simulink model "afe_dqctrl_inv_psm"  (R2026a)
settings: Solver=ode23t  StopTime=simlength  FixedStep=tc  MaxStep=glb_time.tc  RelTol=1e-4
values from neighbouring files (symbols this model uses):
  afe_ctrl = ctrl_afe_setup(glb_time.ts_afe, grid_emu.omega_grid_nom)    [init_model.m]
  afe_pwm_phase_shift_mod1 = 0    [init_model.m]
  CTRPIFF_CLIP_RELEASE = 0.001    [init_model.m]
  filters = setup_global_filters(glb_time.ts_afe, glb_time.ts_inv, glb_time.ts_dab, glb_time.tc)    [init_model.m]
  glb_time = timing_setup(fpwm_afe, trgo_afe, fpwm_inv, trgo_inv, fpwm_single_phase_inv, trgo_single_phase_inv, fpwm_dab, trgo_dab,      fpwm_psfbc, trgo_psfbc, fpwm_isop_rail, trgo_isop_rail, fpwm_cllc, trgo_cllc, t_measure, tc_factor, tc_decimation, delay_pwm, dead_time_afe,      dead_time_inv, dead_time_single_phase_inv, dead_time_dab, dead_time_psfbc, dead_time_isop_rail, dead_time_cllc)    [init_model.m]
  grid_emu = grid_three_phase_emulator('Dyn11', delta_star, grid_nominal_power, application_voltage, us1, us2, fgrid,                  eq_grid_inductance, eq_grid_resistance, eta, ucc, i1m, p_iron, n1, n2, core_area, core_length, mur,                  up_xi_pu_ref, up_eta_pu_ref, un_xi_pu_ref, un_eta_pu_ref)    [init_model.m]
  heatsink = liquid_cooled_plate_2kw_setup(weight, no_weight, cp_al, heat_capacity_hs, thermal_conductivity_al,      Rth_switch_HA, Rth_mosfet_HA, Rth_diode_HA, Tambient, DThs_init)    [init_model.m]
  inv_pwm_phase_shift_mod1 = 0    [init_model.m]
  ki_align = 18    [init_model.m]
  kp_align = 0.25    [init_model.m]
  lim_down_align = -0.05    [init_model.m]
  lim_up_align = 0.05    [init_model.m]
  omega_m_sim = psm.omega_m_bez    [init_model.m]
  psm = psm_calculus()    [init_model.m]
  psm_ctrl = ctrl_pmsm_setup(glb_time.ts_inv, psm.omega_bez, u_psm_scale, psm.Jm_norm)    [init_model.m]
  simlength = 1.75    [init_model.m]
  Tambient = 40    [init_model.m]
  time_gain_afe_module_1 = 1.0002    [init_model.m]
  time_gain_inv_module_2 = 1.001    [init_model.m]
  time_start_motor_control = 0.25    [init_model.m]
  torque_overload_factor = 1.15    [init_model.m]
  u_cm_comp_mod1 = 0    [init_model.m]
  u_psm_scale_ekf = sqrt(3)/2 * 2/3 * hwdata.inv.udc_nom/psm.ubez    [init_model.m]
undefined symbols (not defined in the file or in its folder): hwdata, igbt, magnitude, omega_m_bez, rpm_base, torque_base
libraries: fl_lib x99, nesl_utility x96, igbt_simple_lib x12, single_phase_transformer_lib x3, threephase_inductor_lib x2, dclink_for_two_levels x2, three_phase_pwm_modulator x2, cstblocks_lti x2, discrete_time_low_pass_filter x1, lithium_ion_battery x1, three_phase_voltage_with_frt_emulator x1, simple_flexible_shaft x1
(part 1 of 9)
settings Model: Creator=dbagn  LastModifiedBy=d.bagnara
settings SolverCC: NumberNewtonIterations=3.0  ZeroCrossControl=DisableAll  SolverResetMethod=Robust
settings SFSimCC: CustomCodeUndefinedFunction=ThrowError  DefaultCustomCodeDeterministicFunctions=All
settings SFSimCC: SimCustomHeaderCode=|
  | #include "rpi.h"
  | #include "rpi_simulink.h"
  | #include "bemf_obsv_load_est.h"
  | #include "bemf_obsv_load_est_simulink.h"
  | #include "dqpll_grid.h"
  | #include "dsmavgflt.h"
  | #include "bemf_obsv.h"
  | #include "bemf_obsv_simulink.h"
  | #include "mavgflt.h"
  | #include "mavgflt_simulink.h"
  | #include "mavgflts.h"
  | #include "mavgflts_simulink.h"
  | #include "sv_pwm_cm.h"
  | #include "dsmavgflt_simulink.h"
  | #include "linear_double_integrator_observer_simulink.h"
  | #include "sv_pwm_cm_simulink.h"
  | #include "dqvector_pi.h"
  | #include "dqpll_grid_simulink.h"
  | #include "first_harmonic_tracker.h"
  | #include "dqvector_pi_simulink.h"
  | #include "first_harmonic_tracker_simulink.h"
  | #include "dqpll_thyr.h"
  | #include "sv_pwm_simulink.h"
  | #include "sv_pwm.h"
  | #include "dqpll_thyr_simulink.h"
  | #include "linear_double_integrator_observer.h"
  | #include "math_f.h"
settings SFSimCC: SimUserSources=|
  | "rpi.c"
  | "rpi_simulink.c"
  | "mavgflt_simulink.c"
  | "mavgflt.c"
  | "mavgflts_simulink.c"
  | "mavgflts.c"
  | "dsmavgflt_simulink.c"
  | "dsmavgflt.c"
  | "bemf_obsv_simulink.c"
  | "bemf_obsv.c"
  | "bemf_obsv_load_est_simulink.c"
  | "bemf_obsv_load_est.c"
  | "dqvector_pi.c"
  | "dqvector_pi_simulink.c"
  | "sv_pwm_simulink.c"
  | "sv_pwm.c"
  | "first_harmonic_tracker_simulink.c"
  | "first_harmonic_tracker.c"
  | "dqpll_thyr_simulink.c"
  | "dqpll_thyr.c"
  | "dqpll_grid_simulink.c"
  | "dqpll_grid.c"
  | "linear_double_integrator_observer_simulink.c"
  | "linear_double_integrator_observer.c"
  | "sv_pwm_cm_simulink.c"
  | "sv_pwm_cm.c"
settings SFSimCC: SimUserIncludeDirs=|
  | include
  | src
settings SimscapeCC: SimscapeNominalValues="[{\"value\":\"1\",\"unit\":\"A\"},{\"value\":\"1\",\"unit\":\"bar\"},{\"value\":\"1\",\"unit\":\"cm^2\"},{\"value\":\"1\",\"unit\":\"cm^3/s\"},{\"value\":\"1\",\"unit\":\"kJ/kg\"},{\"value\":\"1\",\"unit\":\"kW\"},{\"value\":\"1\",\"unit\":\"l\"},{\"value\":\"1\",\"unit\":\"N\"},{\"value\":\"1\",\"unit\":\"N*m\"},{\"value\":\"1\",\"unit\":\"V\"}]"  SimscapeLogType=none  SimscapeLogDataHistory=5000.0

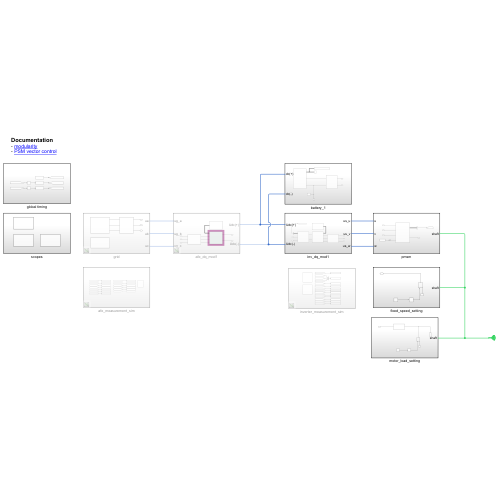
[thumbnail: Simulink's stored preview of the top-level diagram]
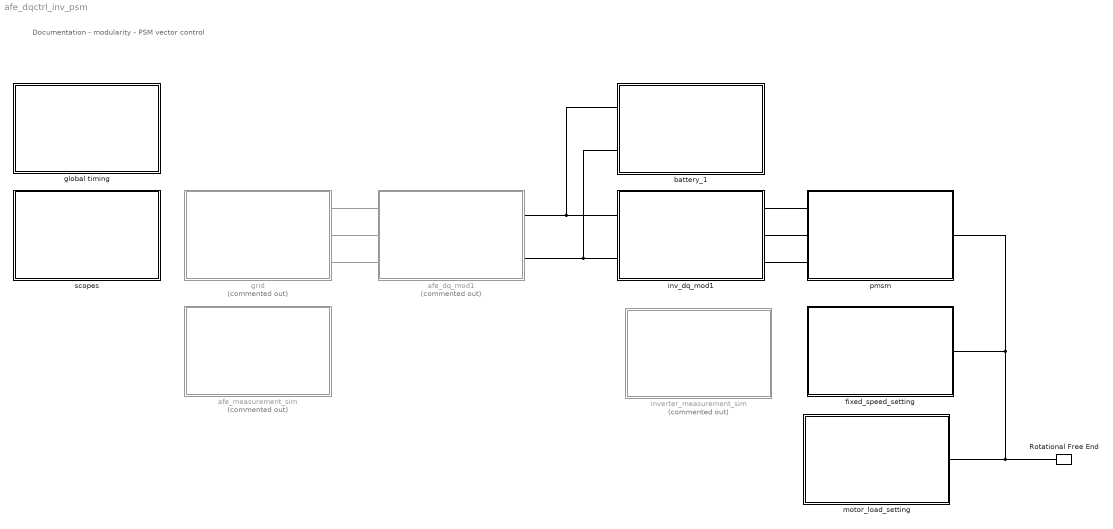
== system afe_dqctrl_inv_psm ==
  note: Documentation
      | - modularity
      | - PSM vector control
  Rotational Free End : fl_lib/Mechanical/Rotational Elements/Rotational Free End  w_specify=off  w_priority=None  w=0 rad/s  w_nominal_specify=off  w_nominal_value=1  w_nominal_unit=rad/s
  afe_dq_mod1 : Subsystem  Commented=on
  afe_measurement_sim : Subsystem  Commented=on
  battery_1 : Subsystem
  fixed_speed_setting : Subsystem
  global timing : Subsystem
  grid : Subsystem  Commented=on
  inv_dq_mod1 : Subsystem
  inverter_measurement_sim : Subsystem  Commented=on
  motor_load_setting : Subsystem
  pmsm : Subsystem
  scopes : Subsystem
  connections:
  pmsm/RConn1 -- motor_load_setting/LConn1 -- Rotational Free End/LConn1 -- fixed_speed_setting/LConn1
  afe_dq_mod1/LConn1 -- grid/RConn1
  afe_dq_mod1/LConn3 -- grid/RConn3
  afe_dq_mod1/LConn2 -- grid/RConn2
  inv_dq_mod1/RConn2 -- pmsm/LConn2
  inv_dq_mod1/RConn1 -- pmsm/LConn1
  inv_dq_mod1/RConn3 -- pmsm/LConn3
  inv_dq_mod1/LConn1 -- afe_dq_mod1/RConn1 -- battery_1/RConn1
  inv_dq_mod1/LConn2 -- afe_dq_mod1/RConn2 -- battery_1/RConn2

== system afe_dqctrl_inv_psm/afe_dq_mod1 ==
  AFE_control : Subsystem
  LCL_filter : Subsystem
  afe : Subsystem
  ug_a : PMIOPort  Side=Left
  ug_b : PMIOPort  Port=2  Side=Left
  ug_c : PMIOPort  Port=3  Side=Left
  Udc(+) : PMIOPort  Port=4  Side=Right
  Udc(-) : PMIOPort  Port=5  Side=Right
  wires:
  AFE_control/1(dabc_out) -> afe/1(dabc)
  connections:
  Udc(-)/RConn1 -- afe/RConn2
  Udc(+)/RConn1 -- afe/RConn1
  LCL_filter/LConn1 -- afe/LConn1
  LCL_filter/LConn2 -- afe/LConn2
  LCL_filter/LConn3 -- afe/LConn3
  ug_a/RConn1 -- LCL_filter/RConn1
  ug_b/RConn1 -- LCL_filter/RConn2
  ug_c/RConn1 -- LCL_filter/RConn3

== system afe_dqctrl_inv_psm/afe_measurement_sim ==
  From6 : From  Commented=on  GotoTag=ileg_dc_afe_mod1
  To Workspace : ToWorkspace  VariableName=t_tc_sim  SampleTime=glb_time.tc
      settings: MaxDataPoints=glb_time.Nc
  To Workspace10 : ToWorkspace  VariableName=P1n_sim  SampleTime=glb_time.ts_afe
      settings: MaxDataPoints=glb_time.Ns_afe
  To Workspace12 : ToWorkspace  Commented=on  VariableName=ileg_dc_afe_sim_mod1  SampleTime=glb_time.tc
      settings: MaxDataPoints=glb_time.Nc
  To Workspace2 : ToWorkspace  VariableName=ic_dclink_sim_mod1  SampleTime=glb_time.tc
      settings: MaxDataPoints=glb_time.Nc
  To Workspace22 : ToWorkspace  VariableName=ig_abc_sim  SampleTime=glb_time.tc
      settings: MaxDataPoints=glb_time.Nc
  To Workspace23 : ToWorkspace  VariableName=ug_abc_sim  SampleTime=glb_time.tc
      settings: MaxDataPoints=glb_time.Nc
  To Workspace3 : ToWorkspace  VariableName=udc_dclink_sim_mod1  SampleTime=glb_time.tc
      settings: MaxDataPoints=glb_time.Nc
  To Workspace4 : ToWorkspace  VariableName=ig_abc_sim_mod1  SampleTime=glb_time.tc
      settings: MaxDataPoints=glb_time.Nc
  To Workspace5 : ToWorkspace  VariableName=vg_abc_sim_mod1  SampleTime=glb_time.tc
      settings: MaxDataPoints=glb_time.Nc
  To Workspace6 : ToWorkspace  VariableName=is_abc_sim_mod1  SampleTime=glb_time.tc
      settings: MaxDataPoints=glb_time.Nc
  To Workspace7 : ToWorkspace  VariableName=Q1n_sim  SampleTime=glb_time.ts_afe
      settings: MaxDataPoints=glb_time.Ns_afe
  To Workspace8 : ToWorkspace  VariableName=Q1p_sim  SampleTime=glb_time.ts_afe
      settings: MaxDataPoints=glb_time.Ns_afe
  To Workspace9 : ToWorkspace  VariableName=P1p_sim  SampleTime=glb_time.ts_afe
      settings: MaxDataPoints=glb_time.Ns_afe
  igbt_power_losses : Subsystem
  wires:
  [time_master] -> To Workspace/1
  [Q1n_global] -> To Workspace7/1
  [Q1p_global] -> To Workspace8/1
  [P1p_global] -> To Workspace9/1
  [P1n_global] -> To Workspace10/1
  [ug_abc] -> To Workspace23/1
  [ig_abc] -> To Workspace22/1
  [ug_abc_pu_mod1] -> To Workspace5/1
  [ig_abc_pu_mod1] -> To Workspace4/1
  From6/1 -> To Workspace12/1
  [udc_mod1] -> To Workspace3/1
  [ic_dclink_mod1] -> To Workspace2/1
  [is_abc_pu_mod1] -> To Workspace6/1

== system afe_dqctrl_inv_psm/battery_1 ==
  Electrical Reference : fl_lib/Electrical/Electrical Elements/Electrical Reference
  Solver Configuration : nesl_utility/Solver Configuration  PhysicalDomain=network_engine_domain  SubClassName=solver  LeftPortType=input  RightPortType=generic  Tones=[]  Harmonics=[]  SimulateNoise=off  Profile=off  UseLocalSampling=off  EnableSwitchedLinearOptims=on  FrequencyDomain=off  UseCCode=off  RelTol=0.001  AbsTol=0.001  MinStep=1e-09  ToWorkspace=off  RevertToSquareIcSolve=off  NumHomotopyIterations=100  PhasorMode=off  PhasorModeNumHarmonics=1  ConsistencySolver=NEWTON_FTOL  CanonicalOrdering=UNORDERED  OptimizeIntermediates=UNOPTIMIZED  IndexReductionMethod=DerivativeReplacement  DoDC=on  ResidualTolerance=1e-09  ConsistencyTolSource=GLOBAL  ConsistencyAbsTol=0.001  ConsistencyRelTol=0.001  ConsistencyTolFactor=0.001  UseLocalSolver=on  LocalSolverChoice=NE_BACKWARD_EULER_ADVANCER  ResolveIndetEquations=on  FunctionEvalNumThread=1  LocalSolverSampleTime=glb_time.tc  DoFixedCost=on  MaxNonlinIter=nonlinear_iterations  MaxModeIter=2  ComputeImpulses=off  ImpulseIterations=2  LinearAlgebra=auto  LinearAlgebraNumThread=0  EquationFormulation=NE_TIME_EF  DelaysMemoryBudget=1024  AutomaticFiltering=on  FilteringTimeConstant=0.001  PartitionStorageMethod=AS_NEEDED  PartitionMemoryBudget=1024  PartitionMethod=ROBUST  MultibodyUseLocalSolver=off  MultibodyLocalSolverChoice=ODE1  MultibodyLocalSolverSampleTime=0.001
  To Workspace14 : ToWorkspace  VariableName=battery_1_data_sim  SampleTime=glb_time.tc
      settings: MaxDataPoints=glb_time.Nc  Decimation=glb_time.decimation_tc
  lithium ion battery : Scope
      settings: ActiveDisplayYMinimum=-808.27997881012811  ActiveDisplayYMaximum=1287.7546757937268  DataLoggingVariableName=ScopeData3
  lithium_ion_battery : lithium_ion_battery/lithium_ion_battery  Q=lithium_ion_battery_1.Q  number_of_cells=lithium_ion_battery_1.number_of_cells  E_1=lithium_ion_battery_1.E_1  E0=lithium_ion_battery_1.E0  E1=lithium_ion_battery_1.E1  E2=lithium_ion_battery_1.E2  E3=lithium_ion_battery_1.E3  Elog=lithium_ion_battery_1.Elog  R0=lithium_ion_battery_1.R0  R1=lithium_ion_battery_1.R1  C1=lithium_ion_battery_1.C1  M=lithium_ion_battery_1.M  alpha=lithium_ion_battery_1.alpha  soc_init=lithium_ion_battery_1.soc_init  ts_battery=glb_time.ts_dab  q1Kalman=lithium_ion_battery_1.q1Kalman  q2Kalman=lithium_ion_battery_1.q2Kalman  q3Kalman=lithium_ion_battery_1.q3Kalman  rKalman=lithium_ion_battery_1.rKalman  tc=glb_time.tc  enable_white_noise_m=0
  single_phase_ui_measure : Subsystem
  dc(+) : PMIOPort  Side=Right
  dc(-) : PMIOPort  Port=2  Side=Right
  wires:
  lithium_ion_battery/1 -> To Workspace14/1, lithium ion battery/1
  connections:
  Solver Configuration/RConn1 -- lithium_ion_battery/RConn2 -- single_phase_ui_measure/LConn2 -- Electrical Reference/LConn1
  single_phase_ui_measure/RConn1 -- dc(+)/RConn1
  single_phase_ui_measure/LConn1 -- lithium_ion_battery/RConn1
  dc(-)/RConn1 -- single_phase_ui_measure/RConn2

== system afe_dqctrl_inv_psm/fixed_speed_setting ==
  Ideal Angular Velocity Source : fl_lib/Mechanical/Mechanical Sources/Ideal Angular Velocity Source
  Mechanical Rotational Reference : fl_lib/Mechanical/Rotational Elements/Mechanical Rotational Reference
  PS Step1 : fl_lib/Physical Signals/Sources/PS Step  step_time=0.025 s  initial_value=0 rpm  final_value=rpm_sim rpm
  PS Transfer Function : fl_lib/Physical Signals/Linear Operators/PS Transfer Function  transfer_function_type=foundation.enum.transfer_function_type.lag  T=0.1 s  T1=2 s  T2=1 s  reset_method=foundation.enum.IntegratorResetSpec.None  initial_condition_spec=foundation.enum.IntegratorICSpec.Internal  y0=0 rpm
  shaft : PMIOPort  Side=Left
  connections:
  Mechanical Rotational Reference/LConn1 -- Ideal Angular Velocity Source/RConn2
  PS Step1/RConn1 -- PS Transfer Function/LConn1
  PS Transfer Function/RConn1 -- Ideal Angular Velocity Source/RConn1
  Ideal Angular Velocity Source/LConn1 -- shaft/RConn1

== system afe_dqctrl_inv_psm/global timing ==
  Unit Delay : UnitDelay  SampleTime=glb_time.tc
  Unit Delay1 : UnitDelay  SampleTime=glb_time.tc
  time_afe1 : Subsystem  mask{k=time_gain_afe_module_1}
      mask prompts: k "Time Gain"
      mask Display:
      | disp('time-gen');
      | port_label('input', 1, 'crt');
      | port_label('output', 1, 'tout');
  time_afe3 : Subsystem  mask{k=1}
      mask prompts: k "Time Gain"
      mask Display:
      | disp('time-gen');
      | port_label('output', 1, 'tout');
  time_inv1 : Subsystem  mask{k=time_gain_inv_module_2}
      mask prompts: k "Time Gain"
      mask Display:
      | disp('time-gen');
      | port_label('input', 1, 'crt');
      | port_label('output', 1, 'tout');
  tag scope: time_afe_module_1=global, time_inv_module_1=global, time_master=global
  wires:
  time_afe1/1(Out1) -> [time_afe_module_1]
  time_inv1/1(Out1) -> [time_inv_module_1]
  time_afe3/1(Out1) -> [time_master]
  [local_time_corr_afe1] -> Unit Delay/1
  Unit Delay/1 -> time_afe1/1(correction_time)
  [local_time_corr_inv1] -> Unit Delay1/1
  Unit Delay1/1 -> time_inv1/1(correction_time)

== system afe_dqctrl_inv_psm/grid ==
  grid_emulator : Subsystem
  power meter iec mfunc : Subsystem
  threephase_vi_measures : Subsystem
  ua : PMIOPort  Side=Right
  ub : PMIOPort  Port=2  Side=Right
  uc : PMIOPort  Port=3  Side=Right
  connections:
  threephase_vi_measures/LConn3 -- grid_emulator/RConn3
  threephase_vi_measures/LConn1 -- grid_emulator/RConn1
  threephase_vi_measures/RConn2 -- ub/RConn1
  threephase_vi_measures/LConn2 -- grid_emulator/RConn2
  threephase_vi_measures/RConn1 -- ua/RConn1
  threephase_vi_measures/RConn3 -- uc/RConn1

== system afe_dqctrl_inv_psm/inv_dq_mod1 ==
  Bus Selector : BusSelector  OutputSignals=vdc_pu
  INV_control : Subsystem
  L_filter : Subsystem
  dclink1 : dclink_for_two_levels/dclink  Cdc=hwdata.afe.CFi  Rudc_measure=1e6  Vdc_scale=hwdata.afe.udc_nom
  inverter : Subsystem
  Udc(+) : PMIOPort  Side=Left
  us_u : PMIOPort  Port=2  Side=Right
  us_v : PMIOPort  Port=3  Side=Right
  Udc(-) : PMIOPort  Port=4  Side=Left
  us_w : PMIOPort  Port=5  Side=Right
  tag scope: udc_pu_inv_mod1=global
  wires:
  INV_control/1(duvw_out) -> inverter/1(duvw)
  Bus Selector/1 -> [udc_pu_inv_mod1]  "<vdc_pu>"
  dclink1/1 -> Bus Selector/1
  connections:
  inverter/LConn1 -- L_filter/RConn1
  L_filter/LConn3 -- us_w/RConn1
  inverter/LConn3 -- L_filter/RConn3
  inverter/LConn2 -- L_filter/RConn2
  L_filter/LConn2 -- us_v/RConn1
  L_filter/LConn1 -- us_u/RConn1
  dclink1/LConn1 -- inverter/RConn1
  dclink1/LConn2 -- inverter/RConn2
  Udc(+)/RConn1 -- dclink1/RConn1
  Udc(-)/RConn1 -- dclink1/RConn2

== system afe_dqctrl_inv_psm/inverter_measurement_sim ==
  Bus Creator : BusCreator  Inputs=3
  To Workspace1 : ToWorkspace  VariableName=ud_psm_sim  SampleTime=glb_time.tc
      settings: MaxDataPoints=glb_time.Nc
  To Workspace10 : ToWorkspace  VariableName=rpm_motor_sim  SampleTime=glb_time.tc
      settings: MaxDataPoints=glb_time.Nc
  To Workspace11 : ToWorkspace  VariableName=iuvw_psm_sim  SampleTime=glb_time.tc
      settings: MaxDataPoints=glb_time.Nc
  To Workspace13 : ToWorkspace  VariableName=theta_elec_psm_sim  SampleTime=glb_time.tc
      settings: MaxDataPoints=glb_time.Nc
  To Workspace2 : ToWorkspace  VariableName=uq_psm_sim  SampleTime=glb_time.tc
      settings: MaxDataPoints=glb_time.Nc
  To Workspace3 : ToWorkspace  VariableName=iq_psm_sim  SampleTime=glb_time.tc
      settings: MaxDataPoints=glb_time.Nc
  To Workspace4 : ToWorkspace  VariableName=id_psm_sim  SampleTime=glb_time.tc
      settings: MaxDataPoints=glb_time.Nc
  To Workspace5 : ToWorkspace  VariableName=inverter_voltage_ee_phase_u_sim  SampleTime=glb_time.tc
      settings: MaxDataPoints=glb_time.Nc
  To Workspace6 : ToWorkspace  VariableName=inverter_voltage_ee_phase_v_sim  SampleTime=glb_time.tc
      settings: MaxDataPoints=glb_time.Nc
  To Workspace7 : ToWorkspace  VariableName=psi_r_alpha_psm_sim  SampleTime=glb_time.tc
      settings: MaxDataPoints=glb_time.Nc
  To Workspace8 : ToWorkspace  VariableName=inverter_voltage_ee_phase_w_sim  SampleTime=glb_time.tc
      settings: MaxDataPoints=glb_time.Nc
  To Workspace9 : ToWorkspace  VariableName=psi_r_beta_psm_sim  SampleTime=glb_time.tc
      settings: MaxDataPoints=glb_time.Nc
  igbt_power_losses : Subsystem
  module_1 : Subsystem
  wires:
  [psi_r_alpha_psm] -> To Workspace7/1  "phi_r_alpha_pmsm"
  [psi_r_beta_psm] -> To Workspace9/1  "phi_r_beta_pmsm"
  [rpm_motor] -> To Workspace10/1
  [iv_psm] -> Bus Creator/2  "iv"
  [iw_psm] -> Bus Creator/3  "iw"
  [iu_psm] -> Bus Creator/1  "iu"
  Bus Creator/1 -> To Workspace11/1
  [theta_elec_psm] -> To Workspace13/1  "theta_elec_pmsm"
  [ud_psm] -> To Workspace1/1  "ud_psm"
  [uq_psm] -> To Workspace2/1  "uq_psm"
  [iq_psm] -> To Workspace3/1  "iq_psm"
  [id_psm] -> To Workspace4/1  "id_psm"
  [inverter_voltage_ee_phase_u] -> To Workspace5/1
  [inverter_voltage_ee_phase_v] -> To Workspace6/1
  [inverter_voltage_ee_phase_w] -> To Workspace8/1

== system afe_dqctrl_inv_psm/motor_load_setting ==
  Ideal Torque Source : fl_lib/Mechanical/Mechanical Sources/Ideal Torque Source
  Inertia : fl_lib/Mechanical/Rotational Elements/Inertia  inertia=external_load_inertia kg*m^2  num_ports=foundation.enum.numPorts2.one  w_specify=off  w_priority=High  w=0 rad/s  w_nominal_specify=off  w_nominal_value=1  w_nominal_unit=rad/s  t_specify=off  t_priority=None  t=0 N*m  t_nominal_specify=off  t_nominal_value=1  t_nominal_unit=N*m
  Mechanical Rotational Reference : fl_lib/Mechanical/Rotational Elements/Mechanical Rotational Reference
  PS Step : fl_lib/Physical Signals/Sources/PS Step  step_time=load_step_time s  initial_value=1 N*m  final_value=1 N*m
  PS Transfer Function : fl_lib/Physical Signals/Linear Operators/PS Transfer Function  transfer_function_type=foundation.enum.transfer_function_type.lag  T=1 s  T1=2 s  T2=1 s  reset_method=foundation.enum.IntegratorResetSpec.None  initial_condition_spec=foundation.enum.IntegratorICSpec.Internal  y0=0 N*m
  flexible_shaft : simple_flexible_shaft/flexible_shaft  b1=1  b2=1  J1=1  J2=1  b_displacement=1  k_displacement=1e5
  shaft : PMIOPort  Side=Left
  connections:
  Ideal Torque Source/LConn1 -- flexible_shaft/RConn1 -- Inertia/LConn1
  Ideal Torque Source/RConn2 -- Mechanical Rotational Reference/LConn1
  PS Transfer Function/RConn1 -- Ideal Torque Source/RConn1
  PS Step/RConn1 -- PS Transfer Function/LConn1
  flexible_shaft/LConn1 -- shaft/RConn1

== system afe_dqctrl_inv_psm/pmsm ==
  Bus Selector1 : BusSelector  OutputSignals=omega_mech (rpm)
  Constant : Constant  Value=psm.psi_m
  Simulink-PS Converter3 : nesl_utility/Simulink-PS Converter  PhysicalDomain=network_engine_domain  SubClassName=ps_input  LeftPortType=input  RightPortType=output  PseudoPeriodic=off  Frequencies=[]  NoiseDistribution=none  NoiseParameters=[]  Unit=V*s  AffineConversion=on  FilteringAndDerivatives=provide  SimscapeFilterOrder=1  InputFilterTimeConstant=0.001  UdotUserProvided=0
  synchronous_motor : Subsystem
  u : PMIOPort  Side=Left
  v : PMIOPort  Port=2  Side=Left
  w : PMIOPort  Port=3  Side=Left
  shaft : PMIOPort  Port=4  Side=Right
  tag scope: rpm_motor=global
  wires:
  synchronous_motor/1(motor_data) -> Bus Selector1/1
  Bus Selector1/1 -> [rpm_motor]  "<omega_mech (rpm)>"
  Constant/1 -> Simulink-PS Converter3/1
  connections:
  synchronous_motor/LConn1 -- u/RConn1
  Simulink-PS Converter3/RConn1 -- synchronous_motor/LConn4
  synchronous_motor/LConn3 -- w/RConn1
  synchronous_motor/LConn2 -- v/RConn1
  shaft/RConn1 -- synchronous_motor/RConn1

== system afe_dqctrl_inv_psm/scopes ==
  cable_effects : Subsystem
  grid_afe_side : Subsystem
  machine_side : Subsystem

== system afe_dqctrl_inv_psm/afe_dq_mod1/AFE_control ==
  To Workspace : ToWorkspace  VariableName=afe_ctrl_data_output_mod1  SampleTime=glb_time.ts_afe
      settings: MaxDataPoints=glb_time.Ns_afe
  afe_control : Subsystem
  dabc_out : Outport
  tag scope: local_time_corr_afe1=global
  wires:
  [TRGO_afe_module_1] -> afe_control/Trigger
  [ug_abc_pu_mod1] -> afe_control/1(ug_abc_pu)
  [is_abc_pu_mod1] -> afe_control/4(is_abc_pu)
  [udc_pu_afe_mod1] -> afe_control/2(udc_pu)
  afe_control/1(duvw) -> dabc_out/1
  [ig_abc_pu_mod1] -> afe_control/3(ig_abc_pu)
  [time_afe_module_1] -> afe_control/5(local_time)
  [time_master] -> afe_control/6(master_time)
  [gamma_grid_emulator] -> afe_control/7(grid_phase)
  afe_control/3(m_data) -> To Workspace/1
  afe_control/2(AFE1_local_time_corr) -> [local_time_corr_afe1]

== system afe_dqctrl_inv_psm/afe_dq_mod1/LCL_filter ==
  CFu1 : fl_lib/Electrical/Electrical Elements/Capacitor  c=hwdata.afe.CFu F  r=hwdata.afe.RCFu Ohm  g=0 1/Ohm  i_specify=off  i_priority=None  i=0 A  i_nominal_specify=off  i_nominal_value=1  i_nominal_unit=A  v_specify=off  v_priority=None  v=0 V  v_nominal_specify=off  v_nominal_value=1  v_nominal_unit=V  vc_specify=off  vc_priority=High  vc=0 V  vc_nominal_specify=off  vc_nominal_value=1  vc_nominal_unit=V
  CFu2 : fl_lib/Electrical/Electrical Elements/Capacitor  c=hwdata.afe.CFu F  r=hwdata.afe.RCFu Ohm  g=0 1/Ohm  i_specify=off  i_priority=None  i=0 A  i_nominal_specify=off  i_nominal_value=1  i_nominal_unit=A  v_specify=off  v_priority=None  v=0 V  v_nominal_specify=off  v_nominal_value=1  v_nominal_unit=V  vc_specify=off  vc_priority=High  vc=0 V  vc_nominal_specify=off  vc_nominal_value=1  vc_nominal_unit=V
  CFu3 : fl_lib/Electrical/Electrical Elements/Capacitor  c=hwdata.afe.CFu F  r=hwdata.afe.RCFu Ohm  g=0 1/Ohm  i_specify=off  i_priority=None  i=0 A  i_nominal_specify=off  i_nominal_value=1  i_nominal_unit=A  v_specify=off  v_priority=None  v=0 V  v_nominal_specify=off  v_nominal_value=1  v_nominal_unit=V  vc_specify=off  vc_priority=High  vc=0 V  vc_nominal_specify=off  vc_nominal_value=1  vc_nominal_unit=V
  Inductor : fl_lib/Electrical/Electrical Elements/Inductor  l=1e-6 H  r=0 Ohm  g=1e-9 1/Ohm  i_specify=on  i_priority=High  i=0 A  i_nominal_specify=off  i_nominal_value=1  i_nominal_unit=A  v_specify=off  v_priority=None  v=0 V  v_nominal_specify=off  v_nominal_value=1  v_nominal_unit=V  i_L_specify=off  i_L_priority=High  i_L=0 A  i_L_nominal_specify=off  i_L_nominal_value=1  i_L_nominal_unit=A
  Inductor1 : fl_lib/Electrical/Electrical Elements/Inductor  l=1e-6 H  r=0 Ohm  g=1e-9 1/Ohm  i_specify=on  i_priority=High  i=0 A  i_nominal_specify=off  i_nominal_value=1  i_nominal_unit=A  v_specify=off  v_priority=None  v=0 V  v_nominal_specify=off  v_nominal_value=1  v_nominal_unit=V  i_L_specify=off  i_L_priority=High  i_L=0 A  i_L_nominal_specify=off  i_L_nominal_value=1  i_L_nominal_unit=A
  Inductor2 : fl_lib/Electrical/Electrical Elements/Inductor  l=1e-6 H  r=0 Ohm  g=1e-9 1/Ohm  i_specify=on  i_priority=High  i=0 A  i_nominal_specify=off  i_nominal_value=1  i_nominal_unit=A  v_specify=off  v_priority=None  v=0 V  v_nominal_specify=off  v_nominal_value=1  v_nominal_unit=V  i_L_specify=off  i_L_priority=High  i_L=0 A  i_L_nominal_specify=off  i_L_nominal_value=1  i_L_nominal_unit=A
  threephase inductor : threephase_inductor_lib/threephase inductor  Lp=hwdata.afe.LFu H  L0=hwdata.afe.LFu_cm H  Rp=hwdata.afe.RLFu Ohm  R0=hwdata.afe.RLFu_cm Ohm  Lls=5e-6 H  uu_1_specify=off  uu_1_priority=None  uu_1=0 V  uu_1_nominal_specify=off  uu_1_nominal_value=1  uu_1_nominal_unit=V  uv_1_specify=off  uv_1_priority=None  uv_1=0 V  uv_1_nominal_specify=off  uv_1_nominal_value=1  uv_1_nominal_unit=V  uw_1_specify=off  uw_1_priority=None  uw_1=0 V  uw_1_nominal_specify=off  uw_1_nominal_value=1  uw_1_nominal_unit=V  uu_2_specify=off  uu_2_priority=None  uu_2=0 V  uu_2_nominal_specify=off  uu_2_nominal_value=1  uu_2_nominal_unit=V  uv_2_specify=off  uv_2_priority=None  uv_2=0 V  uv_2_nominal_specify=off  uv_2_nominal_value=1  uv_2_nominal_unit=V  uw_2_specify=off  uw_2_priority=None  uw_2=0 V  uw_2_nominal_specify=off  uw_2_nominal_value=1  uw_2_nominal_unit=V  iu_specify=off  iu_priority=High  iu=0 A  iu_nominal_specify=off  iu_nominal_value=1  iu_nominal_unit=A  iv_specify=off  iv_priority=High  iv=0 A  iv_nominal_specify=off  iv_nominal_value=1  iv_nominal_unit=A  iw_specify=off  iw_priority=High  iw=0 A  iw_nominal_specify=off  iw_nominal_value=1  iw_nominal_unit=A
  threephase_vi_measures_stack : Subsystem
  threephase_vi_measures_stack1 : Subsystem
  us_a : PMIOPort  Side=Left
  ug_a : PMIOPort  Port=2  Side=Right
  us_b : PMIOPort  Port=3  Side=Left
  ug_b : PMIOPort  Port=4  Side=Right
  us_c : PMIOPort  Port=5  Side=Left
  ug_c : PMIOPort  Port=6  Side=Right
  connections:
  CFu1/RConn1 -- CFu3/RConn1 -- CFu2/RConn1
  Inductor/RConn1 -- threephase_vi_measures_stack1/LConn1 -- CFu1/LConn1
  Inductor2/RConn1 -- CFu3/LConn1 -- threephase_vi_measures_stack1/LConn3
  Inductor1/RConn1 -- CFu2/LConn1 -- threephase_vi_measures_stack1/LConn2
  threephase_vi_measures_stack/LConn1 -- us_a/RConn1
  threephase_vi_measures_stack/LConn2 -- us_b/RConn1
  threephase_vi_measures_stack/LConn3 -- us_c/RConn1
  threephase_vi_measures_stack/RConn1 -- threephase inductor/LConn1
  threephase_vi_measures_stack/RConn2 -- threephase inductor/LConn2
  threephase_vi_measures_stack/RConn3 -- threephase inductor/LConn3
  threephase inductor/RConn1 -- Inductor/LConn1
  Inductor1/LConn1 -- threephase inductor/RConn2
  Inductor2/LConn1 -- threephase inductor/RConn3
  ug_a/RConn1 -- threephase_vi_measures_stack1/RConn1
  ug_b/RConn1 -- threephase_vi_measures_stack1/RConn2
  ug_c/RConn1 -- threephase_vi_measures_stack1/RConn3

== system afe_dqctrl_inv_psm/afe_dq_mod1/afe ==
  dabc : Inport
  Bus Selector : BusSelector  OutputSignals=vdc_pu
  Bus Selector1 : BusSelector  OutputSignals=udc,udc_p_gnd,udc_centertap_gnd,udc_n_gnd  OutputAsBus=on
  Bus Selector2 : BusSelector  OutputSignals=udc
  Bus Selector3 : BusSelector  OutputSignals=Cdc1_current
  dclink1 : dclink_for_two_levels/dclink  Cdc=hwdata.afe.CFi  Rudc_measure=1e6  Vdc_scale=hwdata.afe.udc_nom
  sv_pwm : Subsystem
  three_phase_inverter_with_igbt_simple : Subsystem
  us_a : PMIOPort  Side=Left
  us_b : PMIOPort  Port=2  Side=Left
  us_c : PMIOPort  Port=3  Side=Left
  Udc(+) : PMIOPort  Port=4  Side=Right
  Udc(-) : PMIOPort  Port=5  Side=Right
  tag scope: all_voltages_about_dclink=global, ic_dclink_mod1=global, udc_mod1=global, udc_pu_afe_mod1=global
  wires:
  dabc/1 -> sv_pwm/1(duties_uvw)
  sv_pwm/1(gate_cmds) -> three_phase_inverter_with_igbt_simple/1(gate_commands)
  dclink1/1 -> Bus Selector1/1, Bus Selector2/1, Bus Selector3/1, Bus Selector/1
  Bus Selector1/1 -> [all_voltages_about_dclink]
  Bus Selector/1 -> [udc_pu_afe_mod1]  "<vdc_pu>"
  Bus Selector2/1 -> [udc_mod1]  "<udc>"
  Bus Selector3/1 -> [ic_dclink_mod1]  "<Cdc1_current>"
  connections:
  three_phase_inverter_with_igbt_simple/RConn2 -- us_b/RConn1
  dclink1/RConn1 -- Udc(+)/RConn1
  dclink1/RConn2 -- Udc(-)/RConn1
  three_phase_inverter_with_igbt_simple/RConn1 -- us_a/RConn1
  three_phase_inverter_with_igbt_simple/RConn3 -- us_c/RConn1
  dclink1/LConn2 -- three_phase_inverter_with_igbt_simple/LConn2
  dclink1/LConn1 -- three_phase_inverter_with_igbt_simple/LConn1

== system afe_dqctrl_inv_psm/afe_measurement_sim/igbt_power_losses ==
  To Workspace1 : ToWorkspace  VariableName=igbt_ploss_afeQ1_sim  SampleTime=glb_time.tc
      settings: MaxDataPoints=glb_time.Nc
  To Workspace14 : ToWorkspace  VariableName=igbt_current_afeQ1_sim  SampleTime=glb_time.tc
      settings: MaxDataPoints=glb_time.Nc
  To Workspace15 : ToWorkspace  VariableName=igbt_voltage_afeQ1_sim  SampleTime=glb_time.tc
      settings: MaxDataPoints=glb_time.Nc
  To Workspace16 : ToWorkspace  VariableName=igbt_JH_temp_afeQ1_sim  SampleTime=glb_time.tc
      settings: MaxDataPoints=glb_time.Nc
  To Workspace17 : ToWorkspace  VariableName=igbt_HA_temp_afeQ1_sim  SampleTime=glb_time.tc
      settings: MaxDataPoints=glb_time.Nc
  To Workspace18 : ToWorkspace  VariableName=diode_ploss_afeQ1_sim  SampleTime=glb_time.tc
      settings: MaxDataPoints=glb_time.Nc
  To Workspace19 : ToWorkspace  VariableName=diode_JH_temp_afeQ1_sim  SampleTime=glb_time.tc
      settings: MaxDataPoints=glb_time.Nc
  To Workspace20 : ToWorkspace  VariableName=diode_HA_temp_afeQ1_sim  SampleTime=glb_time.tc
      settings: MaxDataPoints=glb_time.Nc
  wires:
  [igbt_JH_temp_afeQ1] -> To Workspace16/1  "igbt_JH_temp_afeQ1"
  [igbt_ploss_afeQ1] -> To Workspace1/1  "igbt_ploss_afeQ1"
  [igbt_HA_temp_afeQ1] -> To Workspace17/1  "igbt_HA_temp_afeQ1"
  [diode_ploss_afeQ1] -> To Workspace18/1  "diode_ploss_afeQ1"
  [igbt_current_afeQ1] -> To Workspace14/1  "igbt_current_afeQ1"
  [diode_JH_temp_afeQ1] -> To Workspace19/1  "diode_JH_temp_afeQ1"
  [igbt_voltage_afeQ1] -> To Workspace15/1  "igbt_voltage_afeQ1"
  [diode_JH_temp_afeQ1] -> To Workspace20/1  "diode_HA_temp_afeQ1"

== system afe_dqctrl_inv_psm/battery_1/single_phase_ui_measure ==
  Bus Creator : BusCreator  Inputs=2
  Current Sensor : fl_lib/Electrical/Electrical Sensors/Current Sensor
  Selector : Selector  InputPortWidth=2  IndexOptions=Index vector (dialog)  Indices=2  OutputSizes=1
  Selector1 : Selector  InputPortWidth=2  IndexOptions=Index vector (dialog)  Indices=1  OutputSizes=1
  Terminator : Terminator
  Terminator1 : Terminator
  Voltage Sensor : fl_lib/Electrical/Electrical Sensors/Voltage Sensor
  dab input modA : Scope  NumInputPorts=2
      settings: SampleTime=glb_time.tc  ActiveDisplayYMinimum=-255.32963750983237  ActiveDisplayYMaximum=161.62478550201376  DataLoggingVariableName=ScopeData2
  iph : nesl_utility/PS-Simulink Converter  PhysicalDomain=network_engine_domain  SubClassName=ps_output  LeftPortType=input  RightPortType=output  PseudoPeriodic=off  Frequencies=[]  VectorFormat=1-D array  Unit=A  AffineConversion=off
  uph : nesl_utility/PS-Simulink Converter  PhysicalDomain=network_engine_domain  SubClassName=ps_output  LeftPortType=input  RightPortType=output  PseudoPeriodic=off  Frequencies=[]  VectorFormat=1-D array  Unit=V  AffineConversion=off
  Udc(+) : PMIOPort  Side=Left
  udc(+) : PMIOPort  Port=2  Side=Right
  Udc(-) : PMIOPort  Port=3  Side=Left
  udc(-) : PMIOPort  Port=4  Side=Right
  tag scope: current_battery_1=global, voltage_battery_1=global
  wires:
  Bus Creator/1 -> Selector/1, Selector1/1  "ui_data"
  iph/1 -> Bus Creator/1  "iph"
  uph/1 -> Bus Creator/2  "uph"
  Selector1/1 -> [current_battery_1], dab input modA/1  "current_battery"
  Selector/1 -> dab input modA/2, [voltage_battery_1]  "voltage_battery"
  [current_battery_1] -> Terminator/1
  [voltage_battery_1] -> Terminator1/1
  connections:
  iph/LConn1 -- Current Sensor/RConn1
  Voltage Sensor/LConn1 -- Current Sensor/LConn1 -- Udc(+)/RConn1
  Current Sensor/RConn2 -- udc(+)/RConn1
  Voltage Sensor/RConn1 -- uph/LConn1
  Voltage Sensor/RConn2 -- Udc(-)/RConn1 -- udc(-)/RConn1

== system afe_dqctrl_inv_psm/global timing/time_afe1 ==
  correction_time : Inport
  Constant : Constant
  Gain : Gain  Gain=k
  Product : Product
  Sum : Sum  Inputs=|++
  time_1 : Clock
  Out1 : Outport
  wires:
  time_1/1 -> Gain/1
  Gain/1 -> Product/1
  Product/1 -> Out1/1
  correction_time/1 -> Sum/1
  Sum/1 -> Product/2
  Constant/1 -> Sum/2

== system afe_dqctrl_inv_psm/global timing/time_afe3 ==
  Gain : Gain  Gain=k
  time_1 : Clock
  Out1 : Outport
  wires:
  Gain/1 -> Out1/1
  time_1/1 -> Gain/1

== system afe_dqctrl_inv_psm/global timing/time_inv1 ==
  correction_time : Inport
  Constant : Constant
  Gain : Gain  Gain=k
  Product : Product
  Sum : Sum  Inputs=|++
  time_1 : Clock
  Out1 : Outport
  wires:
  time_1/1 -> Gain/1
  Gain/1 -> Product/1
  Product/1 -> Out1/1
  correction_time/1 -> Sum/1
  Constant/1 -> Sum/2
  Sum/1 -> Product/2

== system afe_dqctrl_inv_psm/grid/grid_emulator ==
  3ph_Dyg : Subsystem
  Bus Selector : BusSelector  OutputSignals=ua_grid_emu,ub_grid_emu,uc_grid_emu
  Bus Selector1 : BusSelector  OutputSignals=gamma_grid_emulator,omega_grid_emulator
  Controlled Voltage Source : fl_lib/Electrical/Electrical Sources/Controlled Voltage Source
  Controlled Voltage Source1 : fl_lib/Electrical/Electrical Sources/Controlled Voltage Source
  Controlled Voltage Source2 : fl_lib/Electrical/Electrical Sources/Controlled Voltage Source
  Electrical Reference : fl_lib/Electrical/Electrical Elements/Electrical Reference
  Simulink-PS Converter : nesl_utility/Simulink-PS Converter  PhysicalDomain=network_engine_domain  SubClassName=ps_input  LeftPortType=input  RightPortType=output  PseudoPeriodic=off  Frequencies=[]  NoiseDistribution=none  NoiseParameters=[]  Unit=V  AffineConversion=on  FilteringAndDerivatives=provide  SimscapeFilterOrder=1  InputFilterTimeConstant=0.001  UdotUserProvided=0
  Simulink-PS Converter1 : nesl_utility/Simulink-PS Converter  PhysicalDomain=network_engine_domain  SubClassName=ps_input  LeftPortType=input  RightPortType=output  PseudoPeriodic=off  Frequencies=[]  NoiseDistribution=none  NoiseParameters=[]  Unit=V  AffineConversion=on  FilteringAndDerivatives=provide  SimscapeFilterOrder=1  InputFilterTimeConstant=0.001  UdotUserProvided=0
  Simulink-PS Converter2 : nesl_utility/Simulink-PS Converter  PhysicalDomain=network_engine_domain  SubClassName=ps_input  LeftPortType=input  RightPortType=output  PseudoPeriodic=off  Frequencies=[]  NoiseDistribution=none  NoiseParameters=[]  Unit=V  AffineConversion=on  FilteringAndDerivatives=provide  SimscapeFilterOrder=1  InputFilterTimeConstant=0.001  UdotUserProvided=0
  Solver Configuration : nesl_utility/Solver Configuration  PhysicalDomain=network_engine_domain  SubClassName=solver  LeftPortType=input  RightPortType=generic  Tones=[]  Harmonics=[]  SimulateNoise=off  Profile=off  UseLocalSampling=off  EnableSwitchedLinearOptims=on  FrequencyDomain=off  UseCCode=off  RelTol=0.001  AbsTol=0.001  MinStep=1e-09  ToWorkspace=off  RevertToSquareIcSolve=off  NumHomotopyIterations=100  PhasorMode=off  PhasorModeNumHarmonics=1  ConsistencySolver=NEWTON_FTOL  CanonicalOrdering=UNORDERED  OptimizeIntermediates=UNOPTIMIZED  IndexReductionMethod=DerivativeReplacement  DoDC=on  ResidualTolerance=1e-09  ConsistencyTolSource=GLOBAL  ConsistencyAbsTol=0.001  ConsistencyRelTol=0.001  ConsistencyTolFactor=0.001  UseLocalSolver=on  LocalSolverChoice=NE_BACKWARD_EULER_ADVANCER  ResolveIndetEquations=on  FunctionEvalNumThread=1  LocalSolverSampleTime=glb_time.tc  DoFixedCost=on  MaxNonlinIter=nonlinear_iterations  MaxModeIter=2  ComputeImpulses=off  ImpulseIterations=2  LinearAlgebra=auto  LinearAlgebraNumThread=0  EquationFormulation=NE_TIME_EF  DelaysMemoryBudget=1024  AutomaticFiltering=on  FilteringTimeConstant=0.001  PartitionStorageMethod=AS_NEEDED  PartitionMemoryBudget=1024  PartitionMethod=ROBUST  MultibodyUseLocalSolver=off  MultibodyLocalSolverChoice=ODE1  MultibodyLocalSolverSampleTime=0.001
  td2tc_1 : TransferFcn  Denominator=[glb_time.tc 1]
  td2tc_2 : TransferFcn  Denominator=[glb_time.tc 1]
  td2tc_3 : TransferFcn  Denominator=[glb_time.tc 1]
  three_phase_voltage_source_with_frt_emulator : three_phase_voltage_with_frt_emulator/three_phase_voltage_source_with_frt_emulator  nominal_frequency_m=grid_emu.fgrid_nom  nominal_voltage_m=grid_emu.us_primary_nom  Vemu_ref_norm_m=grid_emu.Vemu_ref_norm  vp_xi_pu_m=grid_emu.up_xi_pu_ref  vp_eta_pu_m=grid_emu.up_eta_pu_ref  vn_xi_pu_m=grid_emu.un_xi_pu_ref  vn_eta_pu_m=grid_emu.un_eta_pu_ref  Am=filters.afe.SOF_50Hz.ss_c.A  Bm=filters.afe.SOF_50Hz.ss_c.B  Cm=filters.afe.SOF_50Hz.ss_c.C  enable_frt_1_m=frt_data.enable_frt_1  enable_frt_2_m=frt_data.enable_frt_2  start_time_LVRT_m=frt_data.start_time_LVRT  end_time_LVRT_m=frt_data.end_time_LVRT  deepPOSxi_m=frt_data.deepPOSxi  deepPOSeta_m=frt_data.deepPOSeta  deepNEGxi_m=frt_data.deepNEGxi  deepNEGeta_m=frt_data.deepNEGeta  Amplitude_U_m=frt_data.Amplitude_U  Amplitude_V_m=frt_data.Amplitude_V  Amplitude_W_m=frt_data.Amplitude_W  t_ramp_m=frt_data.t_ramp  Phase_shift_m=frt_data.Phase_shift
  threephase_vi_measures : Subsystem
  u1 : PMIOPort  Side=Right
  u2 : PMIOPort  Port=2  Side=Right
  u3 : PMIOPort  Port=3  Side=Right
  tag scope: omega_grid_emulator=global, phase_grid_emulator=global
  wires:
  Bus Selector1/2 -> [omega_grid_emulator]  "<omega_grid_emulator>"
  Bus Selector1/1 -> [phase_grid_emulator]  "<gamma_grid_emulator>"
  Bus Selector/2 -> td2tc_2/1  "<ub_grid_emu>"
  Bus Selector/3 -> td2tc_3/1  "<uc_grid_emu>"
  three_phase_voltage_source_with_frt_emulator/1 -> Bus Selector1/1, Bus Selector/1
  Bus Selector/1 -> td2tc_1/1  "<ua_grid_emu>"
  td2tc_1/1 -> Simulink-PS Converter/1  "ua(t)"
  td2tc_2/1 -> Simulink-PS Converter1/1  "ub(t)"
  td2tc_3/1 -> Simulink-PS Converter2/1  "uc(t)"
  connections:
  Simulink-PS Converter/RConn1 -- Controlled Voltage Source/RConn1
  Simulink-PS Converter1/RConn1 -- Controlled Voltage Source1/RConn1
  Simulink-PS Converter2/RConn1 -- Controlled Voltage Source2/RConn1
  Electrical Reference/LConn1 -- Controlled Voltage Source/RConn2 -- Controlled Voltage Source1/RConn2 -- Controlled Voltage Source2/RConn2 -- Solver Configuration/RConn1
  3ph_Dyg/RConn1 -- u1/RConn1
  3ph_Dyg/RConn2 -- u2/RConn1
  3ph_Dyg/RConn3 -- u3/RConn1
  3ph_Dyg/LConn1 -- threephase_vi_measures/RConn1
  3ph_Dyg/LConn2 -- threephase_vi_measures/RConn2
  3ph_Dyg/LConn3 -- threephase_vi_measures/RConn3
  Controlled Voltage Source/LConn1 -- threephase_vi_measures/LConn1
  Controlled Voltage Source1/LConn1 -- threephase_vi_measures/LConn2
  Controlled Voltage Source2/LConn1 -- threephase_vi_measures/LConn3

== system afe_dqctrl_inv_psm/grid/power meter iec mfunc ==
  Bus Selector : BusSelector  OutputSignals=Q1p,Q1n,P1n,P1p,U1n,U1p,i_act_1n,i_react_1n,i_act_1p,i_react_1p
  Constant : Constant  Value=glb_time.ts_afe
  Step : Step  Time=0.025  InitialValue=1  FinalValue=0  SampleTime=0
  To Workspace1 : ToWorkspace  VariableName=i_react_1n  SampleTime=glb_time.ts_afe
      settings: MaxDataPoints=glb_time.Ns_afe
  To Workspace2 : ToWorkspace  VariableName=i_react_1p  SampleTime=glb_time.ts_afe
      settings: MaxDataPoints=glb_time.Ns_afe
  To Workspace3 : ToWorkspace  VariableName=i_act_1n  SampleTime=glb_time.ts_afe
      settings: MaxDataPoints=glb_time.Ns_afe
  To Workspace4 : ToWorkspace  VariableName=i_act_1p  SampleTime=glb_time.ts_afe
      settings: MaxDataPoints=glb_time.Ns_afe
  To Workspace5 : ToWorkspace  VariableName=u1p  SampleTime=glb_time.ts_afe
      settings: MaxDataPoints=glb_time.Ns_afe
  To Workspace6 : ToWorkspace  VariableName=u1n  SampleTime=glb_time.ts_afe
      settings: MaxDataPoints=glb_time.Ns_afe
  Zero-Order Hold{,1..5} (6 alike) : ZeroOrderHold  SampleTime=glb_time.ts_afe
  three_phase_power_meter_iec : MATLAB Function  TreatAsAtomicUnit=on  SystemSampleTime=glb_time.ts_afe
  tag scope: P1n_global=global, P1p_global=global, Q1n_global=global, Q1p_global=global
  wires:
  Bus Selector/6 -> To Workspace5/1  "<U1p>"
  Bus Selector/8 -> To Workspace1/1  "<i_react_1n>"
  Bus Selector/10 -> To Workspace2/1  "<i_react_1p>"
  Bus Selector/5 -> To Workspace6/1  "<U1n>"
  Bus Selector/4 -> [P1p_global]  "<P1p>"
  Bus Selector/2 -> [Q1n_global]  "<Q1n>"
  Bus Selector/1 -> [Q1p_global]  "<Q1p>"
  Bus Selector/7 -> To Workspace3/1  "<i_act_1n>"
  Bus Selector/9 -> To Workspace4/1  "<i_act_1p>"
  Bus Selector/3 -> [P1n_global]  "<P1n>"
  three_phase_power_meter_iec/1(m) -> Bus Selector/1
  Zero-Order Hold/1 -> three_phase_power_meter_iec/1(phase)
  Zero-Order Hold2/1 -> three_phase_power_meter_iec/3(i_abc)
  [phase_grid_emulator] -> Zero-Order Hold/1
  Step/1 -> Zero-Order Hold5/1
  Zero-Order Hold3/1 -> three_phase_power_meter_iec/4(omega)
  Zero-Order Hold4/1 -> three_phase_power_meter_iec/5(ts)
  [ug_abc] -> Zero-Order Hold1/1
  Zero-Order Hold5/1 -> three_phase_power_meter_iec/6(enable_time)
  [ig_abc] -> Zero-Order Hold2/1
  [omega_grid_emulator] -> Zero-Order Hold3/1
  Constant/1 -> Zero-Order Hold4/1
  Zero-Order Hold1/1 -> three_phase_power_meter_iec/2(u_abc)

== system afe_dqctrl_inv_psm/grid/threephase_vi_measures ==
  Bus Creator : BusCreator  Inputs=6
  Current Sensor : fl_lib/Electrical/Electrical Sensors/Current Sensor
  Current Sensor1 : fl_lib/Electrical/Electrical Sensors/Current Sensor
  Current Sensor2 : fl_lib/Electrical/Electrical Sensors/Current Sensor
  Electrical Reference1 : fl_lib/Electrical/Electrical Elements/Electrical Reference
  Selector : Selector  InputPortWidth=6  IndexOptions=Index vector (dialog)  Indices=[1 2 3]  OutputSizes=1
  Selector1 : Selector  InputPortWidth=6  IndexOptions=Index vector (dialog)  Indices=[4 5 6]  OutputSizes=1
  Voltage Sensor : fl_lib/Electrical/Electrical Sensors/Voltage Sensor
  Voltage Sensor1 : fl_lib/Electrical/Electrical Sensors/Voltage Sensor
  Voltage Sensor2 : fl_lib/Electrical/Electrical Sensors/Voltage Sensor
  ia_grid : nesl_utility/PS-Simulink Converter  PhysicalDomain=network_engine_domain  SubClassName=ps_output  LeftPortType=input  RightPortType=output  PseudoPeriodic=off  Frequencies=[]  VectorFormat=1-D array  Unit=A  AffineConversion=off
  ib_grid : nesl_utility/PS-Simulink Converter  PhysicalDomain=network_engine_domain  SubClassName=ps_output  LeftPortType=input  RightPortType=output  PseudoPeriodic=off  Frequencies=[]  VectorFormat=1-D array  Unit=A  AffineConversion=off
  ic_grid : nesl_utility/PS-Simulink Converter  PhysicalDomain=network_engine_domain  SubClassName=ps_output  LeftPortType=input  RightPortType=output  PseudoPeriodic=off  Frequencies=[]  VectorFormat=1-D array  Unit=A  AffineConversion=off
  ig_abc/ug_abc : Scope  NumInputPorts=2
      settings: SampleTime=glb_time.tc  ActiveDisplayYMinimum=-728.92703752654245  ActiveDisplayYMaximum=734.90808013997  DataLoggingVariableName=ScopeData2
  ua_grid : nesl_utility/PS-Simulink Converter  PhysicalDomain=network_engine_domain  SubClassName=ps_output  LeftPortType=input  RightPortType=output  PseudoPeriodic=off  Frequencies=[]  VectorFormat=1-D array  Unit=V  AffineConversion=off
  ub_grid : nesl_utility/PS-Simulink Converter  PhysicalDomain=network_engine_domain  SubClassName=ps_output  LeftPortType=input  RightPortType=output  PseudoPeriodic=off  Frequencies=[]  VectorFormat=1-D array  Unit=V  AffineConversion=off
  uc_grid : nesl_utility/PS-Simulink Converter  PhysicalDomain=network_engine_domain  SubClassName=ps_output  LeftPortType=input  RightPortType=output  PseudoPeriodic=off  Frequencies=[]  VectorFormat=1-D array  Unit=V  AffineConversion=off
  Ua : PMIOPort  Side=Left
  ua : PMIOPort  Port=2  Side=Right
  Ub : PMIOPort  Port=3  Side=Left
  ub : PMIOPort  Port=4  Side=Right
  Uc : PMIOPort  Port=5  Side=Left
  uc : PMIOPort  Port=6  Side=Right
  tag scope: ig_abc=global, ug_abc=global
  wires:
  Bus Creator/1 -> Selector1/1, Selector/1  "vi_data"
  Selector/1 -> [ug_abc]
  ib_grid/1 -> Bus Creator/5  "ib"
  ia_grid/1 -> Bus Creator/4  "ia"
  ic_grid/1 -> Bus Creator/6  "ic"
  ua_grid/1 -> Bus Creator/1  "ua"
  ub_grid/1 -> Bus Creator/2  "ub"
  uc_grid/1 -> Bus Creator/3  "uc"
  Selector1/1 -> [ig_abc]
  [ug_abc] -> ig_abc/ug_abc/2  "ug_abc(line)"
  [ig_abc] -> ig_abc/ug_abc/1  "ig_abc(line)"
  connections:
  Current Sensor1/LConn1 -- Ub/RConn1 -- Voltage Sensor1/LConn1
  Electrical Reference1/LConn1 -- Voltage Sensor/RConn2 -- Voltage Sensor2/RConn2 -- Voltage Sensor1/RConn2
  Voltage Sensor/RConn1 -- ua_grid/LConn1
  Current Sensor/RConn2 -- ua/RConn1
  Voltage Sensor1/RConn1 -- ub_grid/LConn1
  Voltage Sensor2/LConn1 -- Current Sensor2/LConn1 -- Uc/RConn1
  Current Sensor/LConn1 -- Ua/RConn1 -- Voltage Sensor/LConn1
  Current Sensor1/RConn2 -- ub/RConn1
  Voltage Sensor2/RConn1 -- uc_grid/LConn1
  ib_grid/LConn1 -- Current Sensor1/RConn1
  ia_grid/LConn1 -- Current Sensor/RConn1
  ic_grid/LConn1 -- Current Sensor2/RConn1
  Current Sensor2/RConn2 -- uc/RConn1

== system afe_dqctrl_inv_psm/inv_dq_mod1/INV_control ==
  inverter_control : Subsystem
  duvw_out : Outport
  tag scope: local_time_corr_inv1=global, master_torque_ref=global
  wires:
  [is_uvw_pu_mod1] -> inverter_control/1(is_uvw)
  [TRGO_inv_module_1] -> inverter_control/Trigger
  [udc_pu_inv_mod1] -> inverter_control/2(udc_pu)
  inverter_control/1(duvw) -> duvw_out/1
  [time_inv_module_1] -> inverter_control/3(local_time)
  [time_master] -> inverter_control/4(master_time)
  inverter_control/2(local_time_corr) -> [local_time_corr_inv1]
  inverter_control/3(master_torque_ref) -> [master_torque_ref]
  [theta_elec_psm] -> inverter_control/5(theta_elec_psm)
  [omega_elec_psm] -> inverter_control/6(omega_elec_psm)

== system afe_dqctrl_inv_psm/inv_dq_mod1/L_filter ==
  Inductor : fl_lib/Electrical/Electrical Elements/Inductor  l=1e-6 H  r=0 Ohm  g=1e-9 1/Ohm  i_specify=off  i_priority=None  i=0 A  i_nominal_specify=off  i_nominal_value=1  i_nominal_unit=A  v_specify=off  v_priority=None  v=0 V  v_nominal_specify=off  v_nominal_value=1  v_nominal_unit=V  i_L_specify=off  i_L_priority=High  i_L=0 A  i_L_nominal_specify=off  i_L_nominal_value=1  i_L_nominal_unit=A
  Inductor1 : fl_lib/Electrical/Electrical Elements/Inductor  l=1e-6 H  r=0 Ohm  g=1e-9 1/Ohm  i_specify=off  i_priority=None  i=0 A  i_nominal_specify=off  i_nominal_value=1  i_nominal_unit=A  v_specify=off  v_priority=None  v=0 V  v_nominal_specify=off  v_nominal_value=1  v_nominal_unit=V  i_L_specify=off  i_L_priority=High  i_L=0 A  i_L_nominal_specify=off  i_L_nominal_value=1  i_L_nominal_unit=A
  Inductor2 : fl_lib/Electrical/Electrical Elements/Inductor  l=1e-6 H  r=0 Ohm  g=1e-9 1/Ohm  i_specify=off  i_priority=None  i=0 A  i_nominal_specify=off  i_nominal_value=1  i_nominal_unit=A  v_specify=off  v_priority=None  v=0 V  v_nominal_specify=off  v_nominal_value=1  v_nominal_unit=V  i_L_specify=off  i_L_priority=High  i_L=0 A  i_L_nominal_specify=off  i_L_nominal_value=1  i_L_nominal_unit=A
  threephase inductor : threephase_inductor_lib/threephase inductor  Lp=hwdata.inv.LFi H  L0=hwdata.inv.LFi_cm H  Rp=hwdata.inv.RLFi Ohm  R0=hwdata.inv.RLFi_cm Ohm  Lls=5e-6 H  uu_1_specify=off  uu_1_priority=None  uu_1=0 V  uu_1_nominal_specify=off  uu_1_nominal_value=1  uu_1_nominal_unit=V  uv_1_specify=off  uv_1_priority=None  uv_1=0 V  uv_1_nominal_specify=off  uv_1_nominal_value=1  uv_1_nominal_unit=V  uw_1_specify=off  uw_1_priority=None  uw_1=0 V  uw_1_nominal_specify=off  uw_1_nominal_value=1  uw_1_nominal_unit=V  uu_2_specify=off  uu_2_priority=None  uu_2=0 V  uu_2_nominal_specify=off  uu_2_nominal_value=1  uu_2_nominal_unit=V  uv_2_specify=off  uv_2_priority=None  uv_2=0 V  uv_2_nominal_specify=off  uv_2_nominal_value=1  uv_2_nominal_unit=V  uw_2_specify=off  uw_2_priority=None  uw_2=0 V  uw_2_nominal_specify=off  uw_2_nominal_value=1  uw_2_nominal_unit=V  iu_specify=off  iu_priority=None  iu=0 A  iu_nominal_specify=off  iu_nominal_value=1  iu_nominal_unit=A  iv_specify=off  iv_priority=None  iv=0 A  iv_nominal_specify=off  iv_nominal_value=1  iv_nominal_unit=A  iw_specify=off  iw_priority=None  iw=0 A  iw_nominal_specify=off  iw_nominal_value=1  iw_nominal_unit=A
  threephase_vi_measures_stack : Subsystem
  us_u : PMIOPort  Side=Left
  uu : PMIOPort  Port=2  Side=Right
  us_v : PMIOPort  Port=3  Side=Left
  uv : PMIOPort  Port=4  Side=Right
  us_w : PMIOPort  Port=5  Side=Left
  uw : PMIOPort  Port=6  Side=Right
  connections:
  threephase_vi_measures_stack/LConn1 -- us_u/RConn1
  threephase_vi_measures_stack/LConn2 -- us_v/RConn1
  threephase_vi_measures_stack/LConn3 -- us_w/RConn1
  threephase inductor/LConn1 -- threephase_vi_measures_stack/RConn1
  threephase inductor/LConn2 -- threephase_vi_measures_stack/RConn2
  threephase inductor/LConn3 -- threephase_vi_measures_stack/RConn3
  threephase inductor/RConn1 -- Inductor/LConn1
  threephase inductor/RConn2 -- Inductor1/LConn1
  threephase inductor/RConn3 -- Inductor2/LConn1
  Inductor/RConn1 -- uu/RConn1
  Inductor1/RConn1 -- uv/RConn1
  Inductor2/RConn1 -- uw/RConn1
